simulink model "CommandInterface"  (R2024b)
settings: Solver=FixedStepDiscrete  StartTime=0.0  StopTime=inf  RelTol=1e-3  EnableMultiTasking=on
values from neighbouring files (symbols this model uses):
  dataType = 'single'    [mcb_pmsm_foc_qep_f28379d_data.m]
  Ts = T_pwm    (= 5e-05)    [mcb_pmsm_foc_qep_f28379d_data.m]
  TSample = 0.1e-3    (= 0.0001)    [Lez_11_DahlinModel_Parameters_Student.m]
libraries: instrumentseriallib x4, simulink x3
settings Model: Creator=The MathWorks, Inc.  LastModifiedBy=leonardo.lodolini
settings SolverCC: AlgebraicLoopSolver=TrustRegion
settings DataIOCC: LimitDataPoints=on  SaveFormat=Array  ReturnWorkspaceOutputs=off
settings OptimizationCC: LifeSpan=1  EfficientTunableParamExpr=on
settings DebuggingCC: UnderspecifiedInitializationDetection=Classic  MergeDetectMultiDrivingBlocksExec=none  SolverPrmCheckMsg=warning  ParameterPrecisionLossMsg=none  UnconnectedInputMsg=warning  UnconnectedOutputMsg=warning  UnconnectedLineMsg=warning  AllowSymbolicDim=off  PregeneratedLibrarySubsystemCodeDiagnostic=none  SFUnexpectedBacktrackingDiag=warning  SFNoUnconditionalDefaultTransitionDiag=warning  SFExecutionAtInitializationDiag=none  ArithmeticOperatorsInVariantConditions=warning
settings HardwareCC: ProdBitPerPointer=32  ProdLargestAtomicFloat=None  ProdIntDivRoundTo=Undefined  ProdEndianess=Unspecified  ProdWordSize=32  ProdHWDeviceType=32-bit Generic
settings ModelReferenceCC: EnableRefExpFcnMdlSchedulingChecks=on  PropagateSignalLabelsOutOfModel=off
settings SFSimCC: SimUseLocalCustomCode=off  MATLABDynamicMemAlloc=off
settings RTWCC: Description=Real-Time Workshop Embedded Coder  SystemTargetFile=ert.tlc  TemplateMakefile=ert_default_tmf  GenerateReport=on  RTWUseLocalCustomCode=off  IncludeHyperlinkInReport=on  LaunchReport=on  GenerateTraceInfo=on  GenerateTraceReport=on  GenerateTraceReportSl=on  GenerateTraceReportSf=on  GenerateTraceReportEml=on  GPUComputeCapability=3.5  DLArmComputeVersion=19.05
settings CodeAppCC: IgnoreCustomStorageClasses=off  StateflowObjectComments=on  InternalIdentifier=Classic
settings ERTTargetCC: MultiwordLength=2048  GenerateSampleERTMain=on  InlinedParameterPlacement=Hierarchical  ERTCustomFileTemplate=example_file_process.tlc  ConvertIfToSwitch=off  SuppressUnreachableDefaultCases=off  DynamicArrayContainerType=coder::array
settings ConfigComp: CovMetricSettings=dw  CovSaveCumulativeToWorkspaceVar=on  CovSaveSingleToWorkspaceVar=on  CovExternalEMLEnable=off  CovSFcnEnable=off

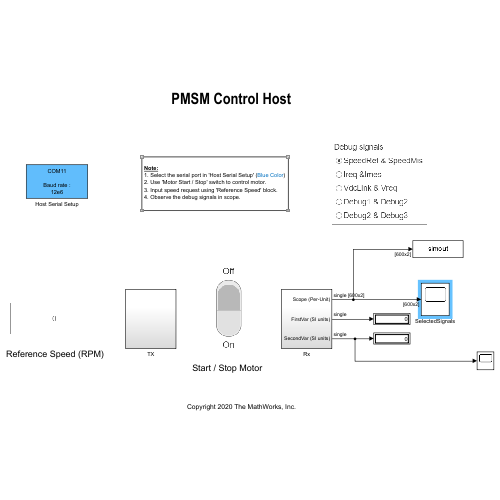
[thumbnail: Simulink's stored preview of the top-level diagram]
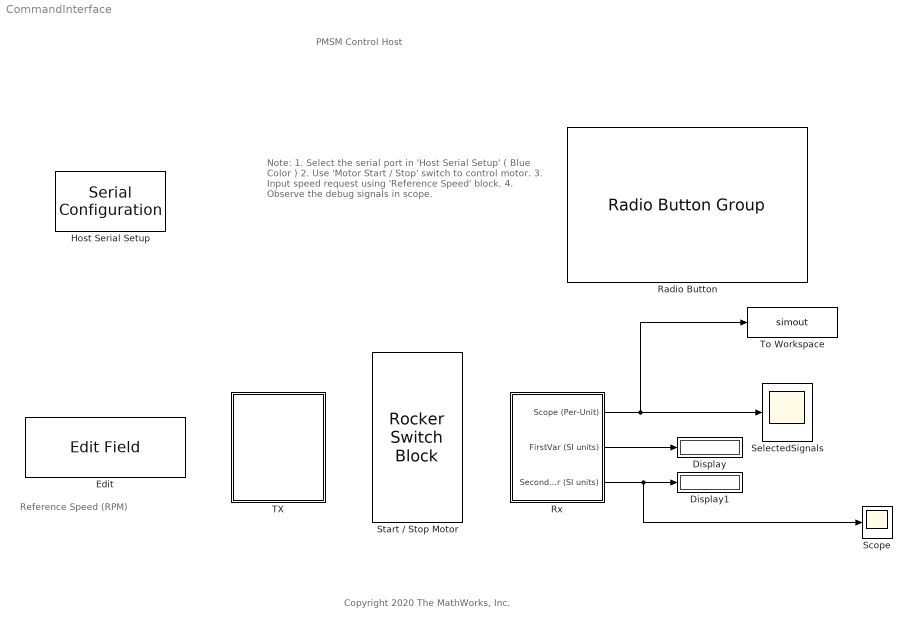
== system CommandInterface ==
  note: PMSM Control Host
  note: Copyright 2020 The MathWorks, Inc.
  note: Note:
      | 1. Select the serial port in 'Host Serial Setup' ( Blue Color )
      | 2. Use 'Motor Start / Stop' switch to control motor.
      | 3. Input speed request using 'Reference Speed' block.
      | 4. Observe the debug signals in scope.
  note: Reference Speed (RPM)
  Display : Display
  Display1 : Display
  Edit : EditField  LabelPosition=Hide  ShowInitialText=on  Alignment=Center
  Host Serial Setup : instrumentseriallib/Serial Configuration  Priority=-99  PortSel=comport  Port=comport  ComPort=comport  BaudRate=12e6  DataBits=8  Parity=none  StopBits=1  ByteOrder=little-endian  FlowControl=none  Timeout=2  SimulateUsing=Interpreted execution  BlockInModel=on  aMode=5
      settings: LibrarySourceBlock=mcbhostblockslib/Host Serial Setup
  Radio Button : RadioButtonGroup  LabelPosition=Hide  SelectedLabel=SpeedRef & SpeedMis  ButtonGroupName=Debug signals
      settings: Values={{'SpeedRef & SpeedMis', 'Ireq &Imes', 'VdcLink & Vreq', 'Debug1 & Debug2', 'Debug2 & Debug3'}, [1 2 3 4 5]}
  Rx : Subsystem
  Scope : Scope
  SelectedSignals : Scope
  "Start / Stop Motor " : RockerSwitchBlock  LabelPosition=Hide
      settings: Values={{'On', 'Off'}, [1 0]}
  TX : Subsystem
  To Workspace : ToWorkspace  VariableName=simout  SampleTime=-1
      settings: Save2DSignal=2-D array (concatenate along first dimension)
  wires:
  Rx/2(FirstVar (SI units)) -> Display/1
  Rx/3(SecondVar (SI units)) -> Scope/1, Display1/1
  Rx/1(Scope (Per-Unit)) -> To Workspace/1, SelectedSignals/1

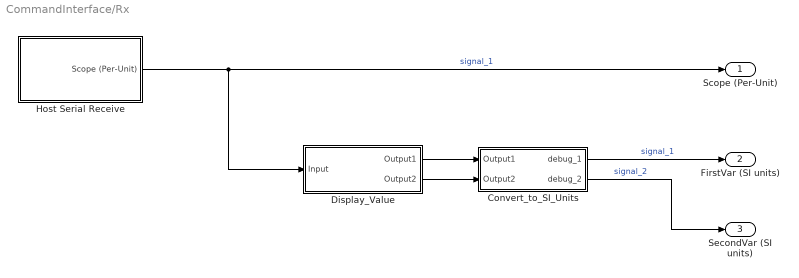
== system CommandInterface/Rx ==
  Convert_to_SI_Units : Subsystem
  Display_Value : MATLAB Function  TreatAsAtomicUnit=on
  Host Serial Receive : Subsystem  Variant=on
  Scope (Per-Unit) : Outport
  FirstVar (SI units) : Outport  Port=2
  SecondVar (SI units) : Outport  Port=3
  wires:
  Host Serial Receive/1(Scope (Per-Unit)) -> Display_Value/1(Input), Scope (Per-Unit)/1  "signal_1"
  Convert_to_SI_Units/1(debug_1) -> FirstVar (SI units)/1  "signal_1"
  Convert_to_SI_Units/2(debug_2) -> SecondVar (SI units)/1  "signal_2"
  Display_Value/1(Output1) -> Convert_to_SI_Units/1(Output1)
  Display_Value/2(Output2) -> Convert_to_SI_Units/2(Output2)

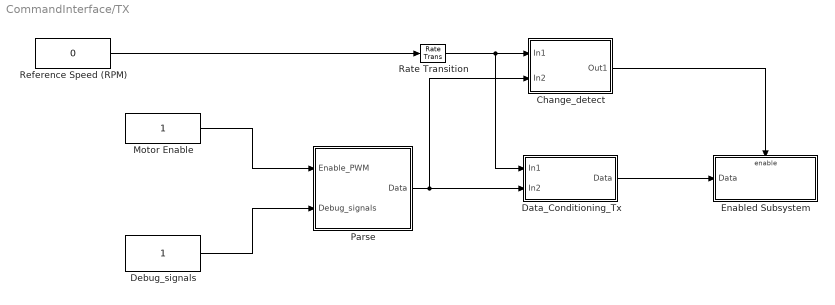
== system CommandInterface/TX ==
  Change_detect : Subsystem
  Data_Conditioning_Tx : Subsystem  Variant=on
  Debug_signals : Constant  OutDataTypeStr=uint16  SampleTime=0.03
  Enabled Subsystem : Subsystem  TreatAsAtomicUnit=on
  Motor Enable : Constant  VectorParams1D=off  OutDataTypeStr=uint16  SampleTime=0.03
  Parse : Subsystem
  Rate Transition : RateTransition  OutPortSampleTime=0.03
  Reference Speed (RPM) : Constant  Value=0  VectorParams1D=off  OutDataTypeStr=single  SampleTime=0.03
  wires:
  Debug_signals/1 -> Parse/2(Debug_signals)
  Data_Conditioning_Tx/1(Data) -> Enabled Subsystem/1(Data)
  Parse/1(Data) -> Data_Conditioning_Tx/2(In2), Change_detect/2(In2)
  Rate Transition/1 -> Data_Conditioning_Tx/1(In1), Change_detect/1(In1)
  Change_detect/1(Out1) -> Enabled Subsystem/Enable
  Motor Enable/1 -> Parse/1(Enable_PWM)
  Reference Speed (RPM)/1 -> Rate Transition/1

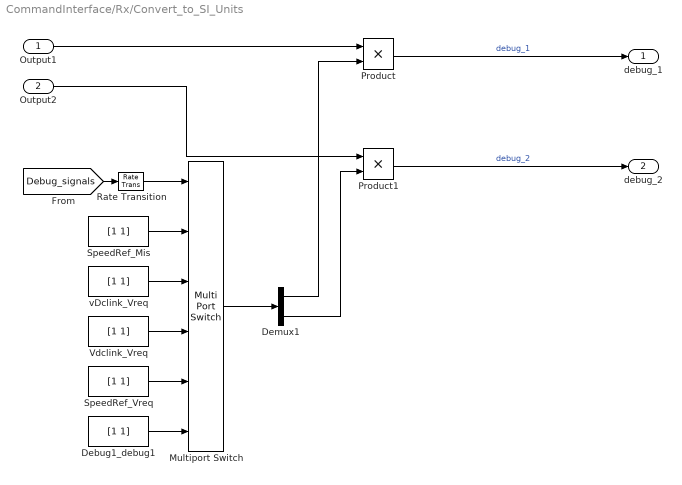
== system CommandInterface/Rx/Convert_to_SI_Units ==
  Output1 : Inport
  Output2 : Inport  Port=2
  Debug1_debug1 : Constant  Value=[1 1]  OutDataTypeStr=single  SampleTime=-1
  Demux1 : Demux  Outputs=2
  Multiport Switch : MultiPortSwitch  Inputs=5  DiagnosticForDefault=Warning  OutDataTypeStr=single  RndMeth=Simplest  SaturateOnIntegerOverflow=off  InputSameDT=off
  Product : Product
  Product1 : Product
  Rate Transition : RateTransition  Deterministic=off
  SpeedRef_Mis : Constant  Value=[1 1]  OutDataTypeStr=single  SampleTime=-1
  SpeedRef_Vreq : Constant  Value=[1 1]  OutDataTypeStr=single  SampleTime=-1
  Vdclink_Vreq : Constant  Value=[1 1]  OutDataTypeStr=single  SampleTime=-1
  vDclink_Vreq : Constant  Value=[1 1]  OutDataTypeStr=single  SampleTime=-1
  debug_1 : Outport
  debug_2 : Outport  Port=2
  wires:
  Product/1 -> debug_1/1  "debug_1"
  Product1/1 -> debug_2/1  "debug_2"
  [Debug_signals] -> Rate Transition/1
  vDclink_Vreq/1 -> Multiport Switch/3
  SpeedRef_Mis/1 -> Multiport Switch/2
  Multiport Switch/1 -> Demux1/1
  SpeedRef_Vreq/1 -> Multiport Switch/5
  Vdclink_Vreq/1 -> Multiport Switch/4
  Demux1/2 -> Product1/2
  Demux1/1 -> Product/2
  Debug1_debug1/1 -> Multiport Switch/6
  Output1/1 -> Product/1
  Output2/1 -> Product1/1
  Rate Transition/1 -> Multiport Switch/1

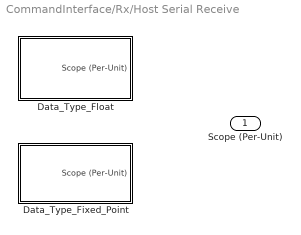
== system CommandInterface/Rx/Host Serial Receive ==
  Data_Type_Fixed_Point : Subsystem  VariantControl=~isequal(dataType, 'single')
  Data_Type_Float : Subsystem  VariantControl=isequal(dataType, 'single')
  Scope (Per-Unit) : Outport

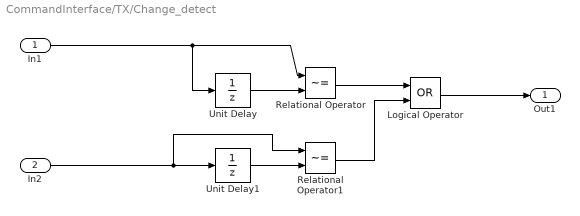
== system CommandInterface/TX/Change_detect ==
  In1 : Inport
  In2 : Inport  Port=2
  Logical Operator : Logic  Operator=OR  AllPortsSameDT=off  OutDataTypeStr=boolean
  Relational Operator : RelationalOperator  Operator=~=  OutDataTypeStr=boolean  InputSameDT=off
  Relational Operator1 : RelationalOperator  Operator=~=  OutDataTypeStr=boolean  InputSameDT=off
  Unit Delay : UnitDelay  InitialCondition=0.5  SampleTime=-1  HasFrameUpgradeWarning=on
  Unit Delay1 : UnitDelay  SampleTime=-1  HasFrameUpgradeWarning=on
  Out1 : Outport  VectorParamsAs1DForOutWhenUnconnected=off
  wires:
  In2/1 -> Relational Operator1/1, Unit Delay1/1
  Relational Operator1/1 -> Logical Operator/2
  Unit Delay1/1 -> Relational Operator1/2
  Unit Delay/1 -> Relational Operator/2
  In1/1 -> Unit Delay/1, Relational Operator/1
  Relational Operator/1 -> Logical Operator/1
  Logical Operator/1 -> Out1/1

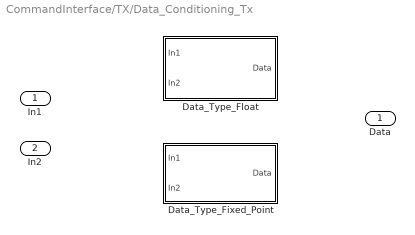
== system CommandInterface/TX/Data_Conditioning_Tx ==
  In1 : Inport
  In2 : Inport  Port=2
  Data_Type_Fixed_Point : Subsystem  VariantControl=~isequal(dataType, 'single')
  Data_Type_Float : Subsystem  VariantControl=isequal(dataType, 'single')
  Data : Outport

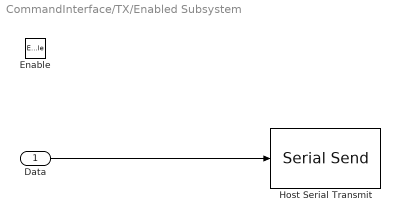
== system CommandInterface/TX/Enabled Subsystem ==
  Data : Inport
  Enable : EnablePort
  Host Serial Transmit : instrumentseriallib/Serial Send  PortSel=comport  Port=comport  ComPort=comport  Header=[]  Terminator=<none>  CustomTerminator=[]  EnableBlockingMode=off  SimulateUsing=Interpreted execution  BlockInModel=on  aMode=5
      settings: LibrarySourceBlock=mcbhostblockslib/Host Serial Transmit
  wires:
  Data/1 -> Host Serial Transmit/1

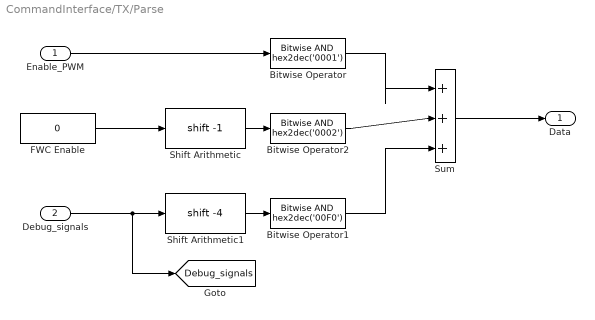
== system CommandInterface/TX/Parse ==
  Enable_PWM : Inport
  Debug_signals : Inport  Port=2
  Bitwise Operator : simulink/Logic and Bit Operations/Bitwise Operator  logicop=AND  UseBitMask=on  BitMask=hex2dec('0001')  BitMaskRealWorld=Stored Integer
  Bitwise Operator1 : simulink/Logic and Bit Operations/Bitwise Operator  logicop=AND  UseBitMask=on  BitMask=hex2dec('00F0')  BitMaskRealWorld=Stored Integer
  Bitwise Operator2 : simulink/Logic and Bit Operations/Bitwise Operator  logicop=AND  UseBitMask=on  BitMask=hex2dec('0002')  BitMaskRealWorld=Stored Integer
  FWC Enable : Constant  Value=0  VectorParams1D=off  OutDataTypeStr=uint16  SampleTime=0.03
  Shift Arithmetic : ArithShift  BitShiftNumber=-1
  Shift Arithmetic1 : ArithShift  BitShiftNumber=-4
  Sum : Sum  Inputs=|+++
  Data : Outport
  tag scope: Debug_signals=global
  wires:
  Bitwise Operator/1 -> Sum/1
  Debug_signals/1 -> [Debug_signals], Shift Arithmetic1/1
  Sum/1 -> Data/1
  Shift Arithmetic1/1 -> Bitwise Operator1/1
  Shift Arithmetic/1 -> Bitwise Operator2/1
  Bitwise Operator1/1 -> Sum/3
  FWC Enable/1 -> Shift Arithmetic/1
  Bitwise Operator2/1 -> Sum/2
  Enable_PWM/1 -> Bitwise Operator/1

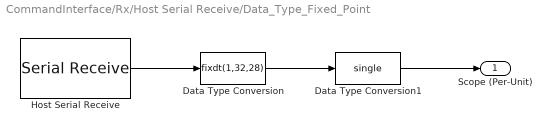
== system CommandInterface/Rx/Host Serial Receive/Data_Type_Fixed_Point ==
  Data Type Conversion : DataTypeConversion  OutDataTypeStr=fixdt(1,32,28)  ConvertRealWorld=Stored Integer (SI)  RndMeth=Simplest  SaturateOnIntegerOverflow=off
  Data Type Conversion1 : DataTypeConversion  OutDataTypeStr=single  RndMeth=Simplest  SaturateOnIntegerOverflow=off
  Host Serial Receive : instrumentseriallib/Serial Receive  PortSel=comport  Port=comport  ComPort=comport  DataType=uint32  SaveDataType=uint8  ToggleHeader=on  Header='SSSS'  ToggleDataSize=on  DataSize=[600 2]  ToggleTerminator=on  Terminator=Custom terminator  CustomTerminator='EEEE'  InputFormat=Row major  EnableBlockingMode=on  ActionDataUnavailable=Output custom value  ActionWhenDataUnavailable=Output custom value  CustomValue=4  SampleTime=600*Ts  SimulateUsing=Interpreted execution  BlockInModel=on  aMode=5
      settings: LibrarySourceBlock=mcbhostblockslib/Host Serial Receive
  Scope (Per-Unit) : Outport
  wires:
  Data Type Conversion/1 -> Data Type Conversion1/1
  Host Serial Receive/1 -> Data Type Conversion/1
  Data Type Conversion1/1 -> Scope (Per-Unit)/1

== system CommandInterface/Rx/Host Serial Receive/Data_Type_Float ==
  Host Serial Receive : instrumentseriallib/Serial Receive  PortSel=comport  Port=comport  ComPort=comport  DataType=single  SaveDataType=uint8  ToggleHeader=on  Header='SSSS'  ToggleDataSize=on  DataSize=[600 2]  ToggleTerminator=on  Terminator=Custom terminator  CustomTerminator='EEEE'  InputFormat=Row major  EnableBlockingMode=on  ActionDataUnavailable=Output custom value  ActionWhenDataUnavailable=Output custom value  CustomValue=4  SampleTime=600*TSample  SimulateUsing=Interpreted execution  BlockInModel=on  aMode=5
      settings: LibrarySourceBlock=mcbhostblockslib/Host Serial Receive
  Scope (Per-Unit) : Outport
  wires:
  Host Serial Receive/1 -> Scope (Per-Unit)/1

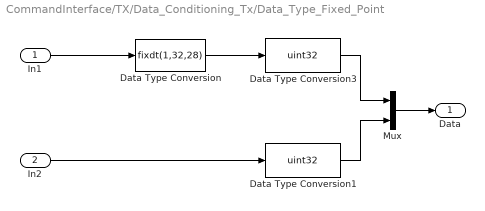
== system CommandInterface/TX/Data_Conditioning_Tx/Data_Type_Fixed_Point ==
  In1 : Inport
  In2 : Inport  Port=2
  Data Type Conversion : DataTypeConversion  OutDataTypeStr=fixdt(1,32,28)  RndMeth=Simplest  SaturateOnIntegerOverflow=off
  Data Type Conversion1 : DataTypeConversion  OutDataTypeStr=uint32  RndMeth=Simplest  SaturateOnIntegerOverflow=off
  Data Type Conversion3 : DataTypeConversion  OutDataTypeStr=uint32  ConvertRealWorld=Stored Integer (SI)  RndMeth=Simplest  SaturateOnIntegerOverflow=off
  Mux : Mux  Inputs=2
  Data : Outport
  wires:
  In1/1 -> Data Type Conversion/1
  Data Type Conversion3/1 -> Mux/1
  Data Type Conversion/1 -> Data Type Conversion3/1
  In2/1 -> Data Type Conversion1/1
  Data Type Conversion1/1 -> Mux/2
  Mux/1 -> Data/1

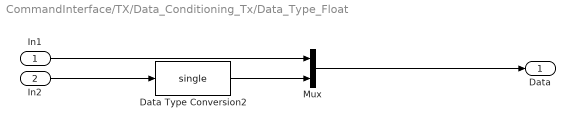
== system CommandInterface/TX/Data_Conditioning_Tx/Data_Type_Float ==
  In1 : Inport
  In2 : Inport  Port=2
  Data Type Conversion2 : DataTypeConversion  OutDataTypeStr=single  RndMeth=Simplest  SaturateOnIntegerOverflow=off
  Mux : Mux  Inputs=2
  Data : Outport
  wires:
  In1/1 -> Mux/1
  Mux/1 -> Data/1
  In2/1 -> Data Type Conversion2/1
  Data Type Conversion2/1 -> Mux/2

== matlab function CommandInterface/Rx/Display_Value ==
  data: Output1 output; Output2 output; Input input
function [ Output1, Output2] = unBuf(Input)
% Unbuffer function
% Outputs first received serial data from buffer for both signals

% Copyright 2020 The MathWorks, Inc.

selSignal= Input(:, 1);
Output1 = selSignal(1,1);
selSignal = Input(:, 2);
Output2 = selSignal(1,1);
end
